simulink model "Regelkreis_T4"  (R2025b)
settings: Solver=ode3  StartTime=0.0  StopTime=5  FixedStep=0.02  RelTol=1e-3
model workspace (MAT data in the model file):
  K_I = 1
  T_1 = [1 1]
settings Model: Creator=ofm31594  LastModifiedBy=jg

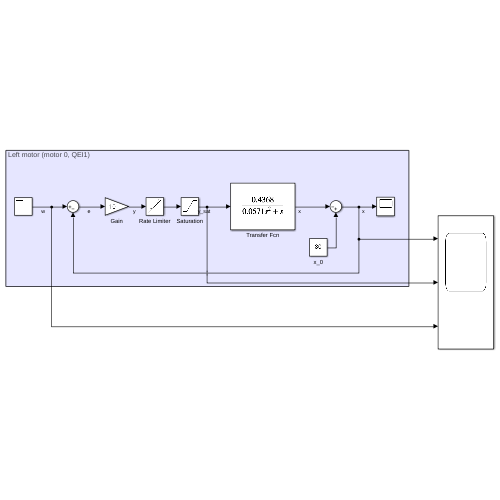
[thumbnail: Simulink's stored preview of the top-level diagram]
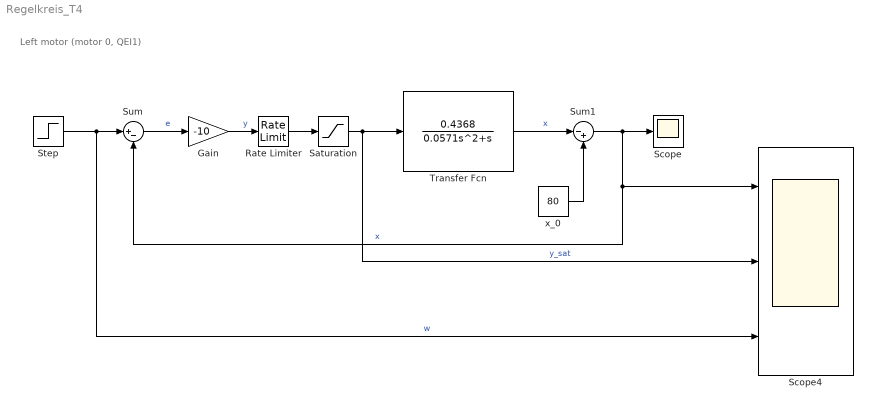
== system Regelkreis_T4 ==
  note: Left motor (motor 0, QEI1)
  Gain : Gain  Gain=-10
  Rate Limiter : RateLimiter  RisingSlewLimit=4/0.02  FallingSlewLimit=-4/0.02  SampleTimeMode=inherited
  Saturation : Saturate  UpperLimit=100  LowerLimit=-100
  Scope : Scope
      settings: ActiveDisplayYMinimum=22.882237420458189  ActiveDisplayYMaximum=86.346418064393532
  Scope4 : Scope  NumInputPorts=3
      settings: ActiveDisplayYMinimum=-115.35662128410816  ActiveDisplayYMaximum=123.92851347601201  DataLoggingVariableName=ScopeData4
  Step : Step  Before=80  After=25  SampleTime=0  VectorParams1D=off  ZeroCross=off
  Sum : Sum  Inputs=|+-
  Sum1 : Sum  Inputs=|-+
  Transfer Fcn : TransferFcn  Numerator=0.4368  Denominator="[ 0.0571 1  0]"
  x_0 : Constant  Value=80
  wires:
  Sum/1 -> Gain/1  "e"
  Gain/1 -> Rate Limiter/1  "y"
  Step/1 -> Scope4/3, Sum/1  "w"
  Sum1/1 -> Scope4/1, Sum/2, Scope/1  "x"
  Transfer Fcn/1 -> Sum1/1  "x"
  x_0/1 -> Sum1/2
  Rate Limiter/1 -> Saturation/1
  Saturation/1 -> Scope4/2, Transfer Fcn/1  "y_sat"
